simulink model "dynamic_of_reaction_wheel_mine"  (R2025a)
settings: Solver=VariableStepAuto  StartTime=0.0  StopTime=100  RelTol=1e-3
InitFcn:
  | run('D:\Work\Personal project\cubli\Matlab sim\Params.m');
values from neighbouring files (symbols this model uses):
  body_accel_gain = 1/IcO_bar    [Params.m]
  bw = 1.06e-5    (= 1.06e-05)    [Params.m]
  cd = 1.70e-8    (= 1.7e-08)    [Params.m]
  gravity_gain = mtot*g*d    [Params.m]
  tau_c = 2.46e-3    (= 0.00246)    [Params.m]
  tau_input = 0    [Params.m]
  w_eps = 0.5    [Params.m]
  wheel_accel_gain = 1/Iwg    (= 8000)    [Params.m]
settings Model: NumberOfSteps=5  Creator=Tran Anh Duy  LastModifiedBy=Tran Anh Duy

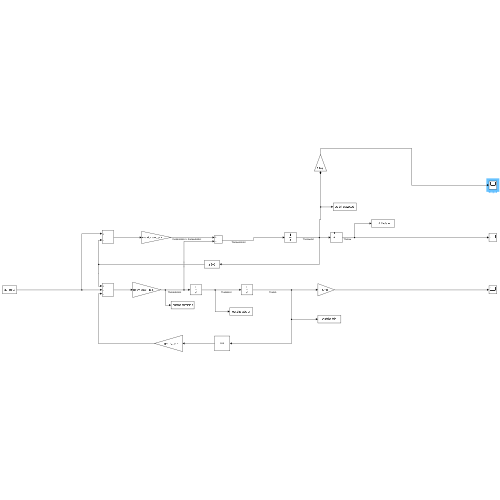
[thumbnail: Simulink's stored preview of the top-level diagram]
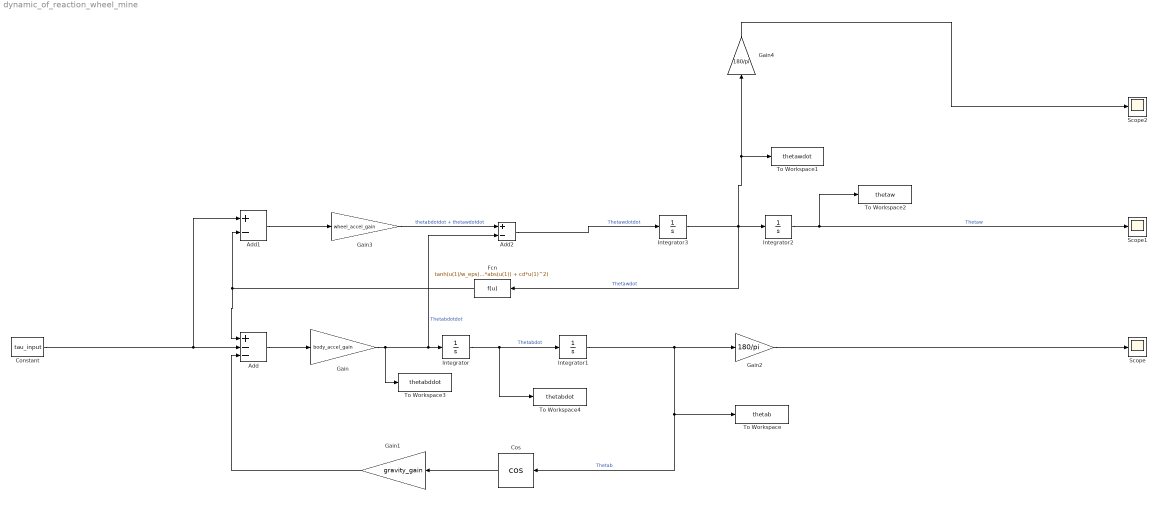
== system dynamic_of_reaction_wheel_mine ==
  Add : Sum  Inputs=+--
  Add1 : Sum  Inputs=+-
  Add2 : Sum  Inputs=+-
  Constant : Constant  Value=tau_input
  Cos : Trigonometry  Operator=cos
  Fcn : Fcn  Expr=tanh(u(1)/w_eps)*(tau_c + bw*abs(u(1)) + cd*u(1)^2)
  Gain : Gain  Gain=body_accel_gain
  Gain1 : Gain  Gain=gravity_gain
  Gain2 : Gain  Gain=180/pi
  Gain3 : Gain  Gain=wheel_accel_gain
  Gain4 : Gain  Gain=180/pi
  Integrator : Integrator
  Integrator1 : Integrator  InitialCondition=45*pi/180
  Integrator2 : Integrator
  Integrator3 : Integrator
  Scope : Scope
      settings: ActiveDisplayYMinimum=-244.71925559248353  ActiveDisplayYMaximum=40.890610031872
  Scope1 : Scope
      settings: ActiveDisplayYMinimum=-3.1325052749787066  ActiveDisplayYMaximum=5.1190465729474406
  Scope2 : Scope
      settings: ActiveDisplayYMinimum=-1032.0434772028864  ActiveDisplayYMaximum=927.47312287227248  DataLoggingVariableName=ScopeData2
  To Workspace : ToWorkspace  VariableName=thetab  SampleTime=-1
  To Workspace1 : ToWorkspace  VariableName=thetawdot  SampleTime=-1
  To Workspace2 : ToWorkspace  VariableName=thetaw  SaveFormat=Timeseries  SampleTime=-1
  To Workspace3 : ToWorkspace  VariableName=thetabddot  SampleTime=-1
  To Workspace4 : ToWorkspace  VariableName=thetabdot  SampleTime=-1
  wires:
  Add/1 -> Gain/1
  Gain/1 -> To Workspace3/1, Add2/2, Integrator/1  "Thetabdotdot"
  Integrator/1 -> To Workspace4/1, Integrator1/1  "Thetabdot"
  Integrator1/1 -> To Workspace/1, Cos/1, Gain2/1  "Thetab"
  Gain1/1 -> Add/3
  Constant/1 -> Add1/1, Add/2
  Integrator3/1 -> Fcn/1, Integrator2/1, Gain4/1, To Workspace1/1  "Thetawdot"
  Integrator2/1 -> To Workspace2/1, Scope1/1  "Thetaw"
  Add1/1 -> Gain3/1
  Cos/1 -> Gain1/1
  Gain2/1 -> Scope/1
  Fcn/1 -> Add/1, Add1/2
  Gain4/1 -> Scope2/1
  Gain3/1 -> Add2/1  "thetabdotdot + thetawdotdot"
  Add2/1 -> Integrator3/1  "Thetawdotdot"
